simulink model "modeloNL1"  (R2025a)
settings: Solver=VariableStepAuto  StartTime=0.0  StopTime=100  FixedStep=0.01  RelTol=1e-3
undefined symbols (not defined in the file): C_alt, C_phi, C_theta, C_vel, INPUTS, Kp, Kp_sas, Kq, Kr, TrimInput, Xe
libraries: slpidlib x9
settings Model: Creator=anade  LastModifiedBy=Kaue

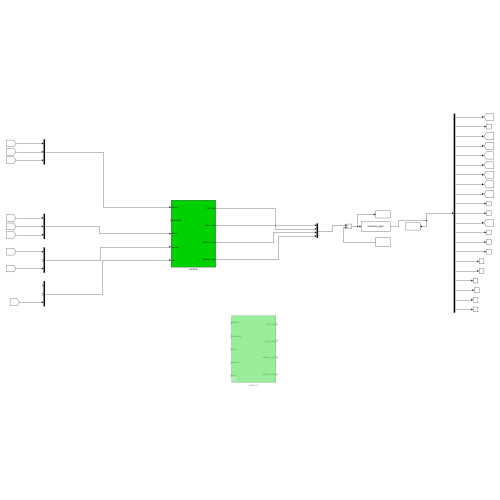
[thumbnail: Simulink's stored preview of the top-level diagram]
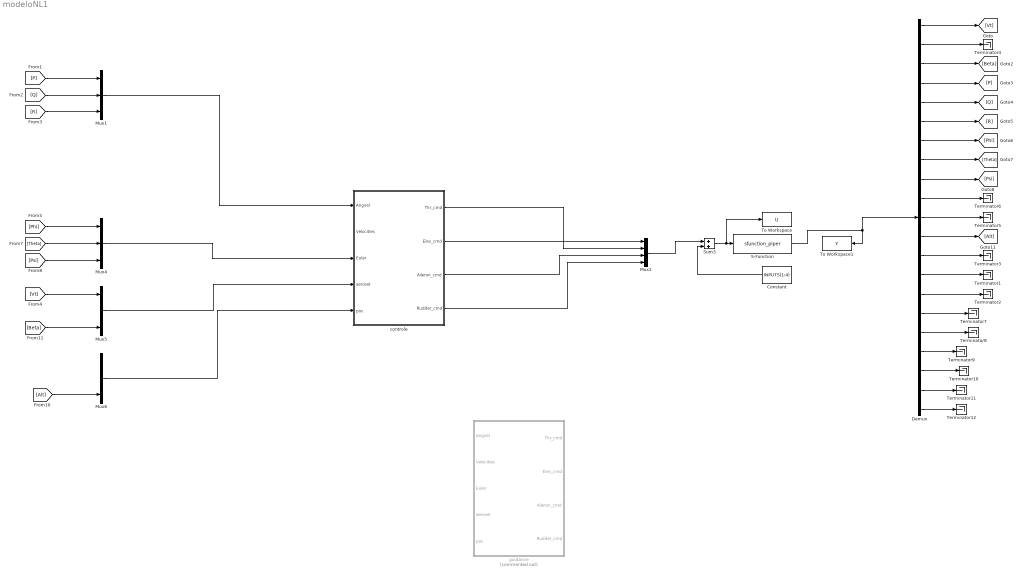
== system modeloNL1 ==
  Constant : Constant  Value=INPUTS(1:4)
  Demux : Demux  Outputs=21
  Mux{1,4..6} (4 alike) : Mux  Inputs=3
  Mux2 : Mux
  S-Function : S-Function  FunctionName=sfunction_piper  Parameters=par_gen,par_aero,par_prop, Xe  SFunctionDeploymentMode=off  EnableBusSupport=off
  Sum3 : Sum
  Terminator{1..12} (12 alike) : Terminator
  To Workspace : ToWorkspace  VariableName=U  SaveFormat=Structure With Time  SampleTime=-1
  To Workspace1 : ToWorkspace  VariableName=Y  SaveFormat=Structure With Time  SampleTime=-1
  controle : Subsystem
  guidance : Subsystem  Commented=on
  wires:
  S-Function/1 -> To Workspace1/1, Demux/1
  Sum3/1 -> To Workspace/1, S-Function/1
  controle/4(Rudder_cmd) -> Mux2/4
  controle/3(Aileron_cmd) -> Mux2/3
  Mux2/1 -> Sum3/1
  Constant/1 -> Sum3/2
  Demux/2 -> Terminator4/1
  Demux/3 -> [Beta]
  Demux/4 -> [P]
  Demux/5 -> [Q]
  Demux/6 -> [R]
  Demux/7 -> [Phi]
  Demux/8 -> [Theta]
  Demux/10 -> Terminator6/1
  Demux/11 -> Terminator5/1
  Demux/13 -> Terminator3/1
  Demux/14 -> Terminator1/1
  Demux/15 -> Terminator2/1
  Demux/1 -> [Vt]
  [Theta] -> Mux4/2
  Mux1/1 -> controle/1(Angvel)
  [Alt] -> Mux6/3
  [P] -> Mux1/1
  Mux4/1 -> controle/3(Euler)
  [R] -> Mux1/3
  [Phi] -> Mux4/1
  Mux6/1 -> controle/5(pos)
  [Q] -> Mux1/2
  Mux5/1 -> controle/4(aerovel)
  [Psi] -> Mux4/3
  [Beta] -> Mux5/3
  Demux/9 -> [Psi]
  [Vt] -> Mux5/1
  Demux/12 -> [Alt]
  controle/2(Elev_cmd) -> Mux2/1
  controle/1(Thr_cmd) -> Mux2/2
  Demux/17 -> Terminator8/1
  Demux/16 -> Terminator7/1
  Demux/19 -> Terminator10/1
  Demux/18 -> Terminator9/1
  Demux/21 -> Terminator12/1
  Demux/20 -> Terminator11/1

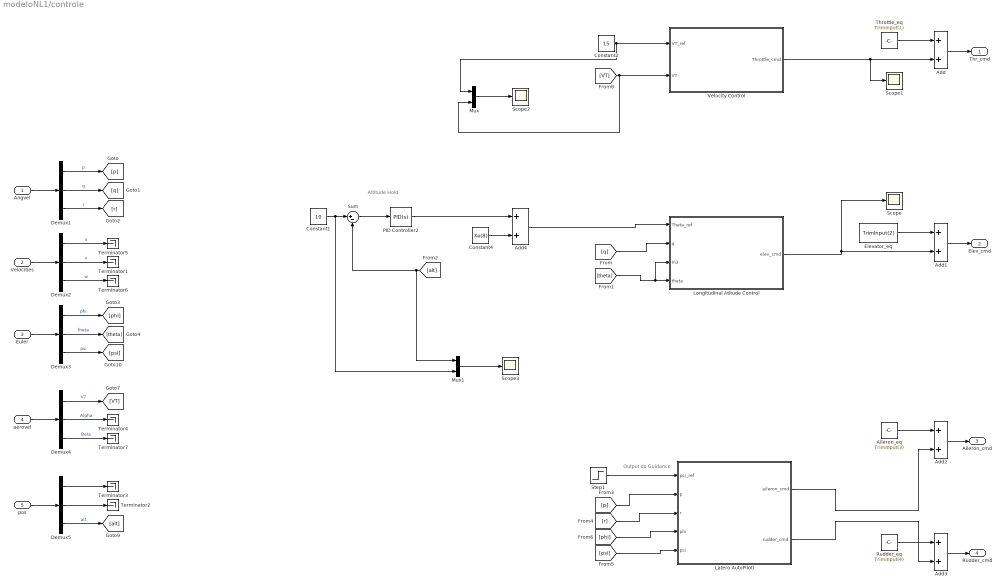
== system modeloNL1/controle ==
  note: Altitude Hold
  note: Output do Guidance
  Angvel : Inport
  Velocities : Inport  Port=2
  Euler : Inport  Port=3
  aerovel : Inport  Port=4
  pos : Inport  Port=5
  Add{,1..4} (5 alike) : Sum
  Aileron_eq : Constant  Value=TrimInput(3)
  Constant1 : Constant  Value=10
  Constant2 : Constant  Value=15
  Constant4 : Constant  Value=Xe(8)
  Demux{1..5} (5 alike) : Demux  Outputs=3
  Elevator_eq : Constant  Value=TrimInput(2)
  Latero AutoPilotl : Subsystem
  Longitudinal Atitude Control : Subsystem
  Mux : Mux  Inputs=2
  Mux1 : Mux  Inputs=2
  PID Controller2 : slpidlib/PID Controller  Controller=PID  Form=Parallel  TimeDomain=Continuous-time  UseExternalTs=off  SampleTime=-1  IntegratorMethod=Forward Euler  FilterMethod=Forward Euler  ControllerParametersSource=internal  P=C_alt.Kp  I=C_alt.Ki  UseKiTs=off  D=C_alt.Kd  UseExternalDerivativeSource=off  N=C_alt.N  UseFilter=on  TunerSelectOption=Transfer Function Based (PID Tuner App)  InitialConditionSource=internal  InitialConditionForIntegrator=0  InitialConditionForFilter=0  DifferentiatorICPrevScaledInput=0  ExternalReset=none  TrackingMode=off  Kt=1  LimitOutput=on  SatLimitsSource=internal  UpperSaturationLimit=0.26  LowerSaturationLimit=-0.17  LinearizeAsGain=on  AntiWindupMode=clamping  Kb=1  LimitIntegrator=off  UpperIntegratorSaturationLimit=inf  LowerIntegratorSaturationLimit=-inf  POutMin=[]  POutMax=[]  IOutMin=[]  IOutMax=[]  DOutMin=[]  DOutMax=[]  NOutMin=[]  NOutMax=[]  SumOutMin=[]  SumOutMax=[]  SaturationOutMin=[]  SaturationOutMax=[]  PParamMin=[]  PParamMax=[]  IParamMin=[]  IParamMax=[]  DParamMin=[]  DParamMax=[]  NParamMin=[]  NParamMax=[]  KbParamMin=[]  KbParamMax=[]  KtParamMin=[]  KtParamMax=[]  KbOutMin=[]  KbOutMax=[]  KtOutMin=[]  KtOutMax=[]  IntegratorOutMin=[]  IntegratorOutMax=[]  FilterOutMin=[]  FilterOutMax=[]  SumI1OutMin=[]  SumI1OutMax=[]  SumI2OutMin=[]  SumI2OutMax=[]  SumI3OutMin=[]  SumI3OutMax=[]  SumI4OutMin=[]  SumI4OutMax=[]  SumDOutMin=[]  SumDOutMax=[]  DifferentiatorOutMin=[]  DifferentiatorOutMax=[]  FilterDiffOutCoefMin=[]  FilterDiffOutCoefMax=[]  ReciprocalOutMin=[]  ReciprocalOutMax=[]  SumDenOutMin=[]  SumDenOutMax=[]  SumNumOutMin=[]  SumNumOutMax=[]  DivideOutMin=[]  DivideOutMax=[]  UdiffTsProdOutMin=[]  UdiffTsProdOutMax=[]  NTsProdOutMin=[]  NTsProdOutMax=[]  UintegralTsProdOutMin=[]  UintegralTsProdOutMax=[]  UngainTsProdOutMin=[]  UngainTsProdOutMax=[]  ClampingZeroOutDataTypeStr=Inherit: Inherit via back propagation  ClampingZeroOutMin=[]  ClampingZeroOutMax=[]  FilterDenConstantOutDataTypeStr=Inherit: Inherit via back propagation  FilterDenConstantOutMin=[]  FilterDenConstantOutMax=[]  PCopyOutDataTypeStr=Inherit: Inherit via back propagation  PCopyOutMin=[]  PCopyOutMax=[]  NCopyOutDataTypeStr=Inherit: Inherit via back propagation  NCopyOutMin=[]  NCopyOutMax=[]  IntegratorContinuousStateAttributes=''  IntegratorStateMustResolveToSignalObject=off  IntegratorRTWStateStorageClass=Auto  FilterContinuousStateAttributes=''  FilterStateMustResolveToSignalObject=off  FilterRTWStateStorageClass=Auto  ParallelPVariant=InternalParameters  IdealPVariant=Disabled  IVariant=InternalParameters  DVariant=InternalParameters  IntegratorVariant=Continuous  SatVariant=Enabled  AWVariant=ContClampingParallel  PCopyVariant=Disabled  TRVariant=Disabled  FdbkBlocksVariant=Forward  IdealPFdbkVariant=Disabled  SatFdbkVariant=Disabled  DerivativeFilterVariant=ContFilter  NVariant=InternalParameters  NCopyVariant=Disabled  FilterICVariant=InternalICsFilter  IntegratorICVariant=InternalICs  ExternalResetVariant=Disabled  TRSumVariant=Passthrough  SumFdbkVariant=Disabled  SumVariant=Sum_PID  TsampFilterVariant=InternalTs  TsampNgainVariant=Passthrough  TsampIntegralVariant=Disabled_SignalSpec  ExternalSaturationOutDataTypeStr=Inherit: Same as second input  DerivativeSourceVariant=ErrorSignal  PreIntVariant=InternalPreInt
  Rudder_eq : Constant  Value=TrimInput(4)
  Scope{,1..3} (4 alike) : Scope
      Scope settings: ActiveDisplayYMinimum=-1E-5  ActiveDisplayYMaximum=0.0001
      Scope1 settings: ActiveDisplayYMinimum=-746.9186  ActiveDisplayYMaximum=116.1605  DataLoggingVariableName=ScopeData2
      Scope2 settings: ActiveDisplayYMinimum=-99.881928520684582  ActiveDisplayYMaximum=101.11428639075469  DataLoggingVariableName=ScopeData4
      Scope3 settings: ActiveDisplayYMinimum=-113.29137312954269  ActiveDisplayYMaximum=148.47510576001991  DataLoggingVariableName=ScopeData6
  Step1 : Step  Time=5  After=deg2rad(45)  SampleTime=0
  Sum : Sum  Inputs=|+-
  Terminator{1..7} (7 alike) : Terminator
  Throttle_eq : Constant  Value=TrimInput(1)
  Velocity Control : Subsystem
  Thr_cmd : Outport
  Elev_cmd : Outport  Port=2
  Aileron_cmd : Outport  Port=3
  Rudder_cmd : Outport  Port=4
  wires:
  Angvel/1 -> Demux1/1
  Velocities/1 -> Demux2/1
  Demux1/1 -> [p]  "p"
  Demux1/2 -> [q]  "q"
  Demux1/3 -> [r]  "r"
  Euler/1 -> Demux3/1
  Demux3/3 -> [psi]  "psi"
  Demux3/1 -> [phi]  "phi"
  Demux3/2 -> [theta]  "theta"
  Demux2/3 -> Terminator6/1  "w"
  Demux2/1 -> Terminator5/1  "u"
  Demux2/2 -> Terminator1/1  "v"
  [theta] -> Longitudinal Atitude Control/3(In3), Longitudinal Atitude Control/4(theta)
  aerovel/1 -> Demux4/1
  Demux4/1 -> [VT]  "VT"
  Demux4/2 -> Terminator4/1  "Alpha"
  Demux4/3 -> Terminator7/1  "Beta"
  [q] -> Longitudinal Atitude Control/2(q)
  [VT] -> Mux/2, Velocity Control/2(VT)
  pos/1 -> Demux5/1
  Demux5/3 -> [alt]  "alt"
  Demux5/2 -> Terminator2/1
  Demux5/1 -> Terminator3/1
  [alt] -> Sum/2, Mux1/1
  [p] -> Latero AutoPilotl/2(p)
  [r] -> Latero AutoPilotl/3(r)
  [psi] -> Latero AutoPilotl/5(psi)
  [phi] -> Latero AutoPilotl/4(phi)
  Constant4/1 -> Add4/2
  Add4/1 -> Longitudinal Atitude Control/1(Theta_ref)
  Step1/1 -> Latero AutoPilotl/1(psi_ref)
  Constant1/1 -> Mux1/2, Sum/1
  Mux/1 -> Scope2/1
  Add1/1 -> Elev_cmd/1
  Longitudinal Atitude Control/1(elev_cmd) -> Scope/1, Add1/2
  Add/1 -> Thr_cmd/1
  Velocity Control/1(Throttle_cmd) -> Scope1/1, Add/2
  Latero AutoPilotl/1(aileron_cmd) -> Add2/2
  Elevator_eq/1 -> Add1/1
  Rudder_eq/1 -> Add3/1
  Aileron_eq/1 -> Add2/1
  Latero AutoPilotl/2(rudder_cmd) -> Add3/2
  Add2/1 -> Aileron_cmd/1
  Add3/1 -> Rudder_cmd/1
  Throttle_eq/1 -> Add/1
  Mux1/1 -> Scope3/1
  Sum/1 -> PID Controller2/1
  PID Controller2/1 -> Add4/1
  Constant2/1 -> Mux/1, Velocity Control/1(VT_ref)

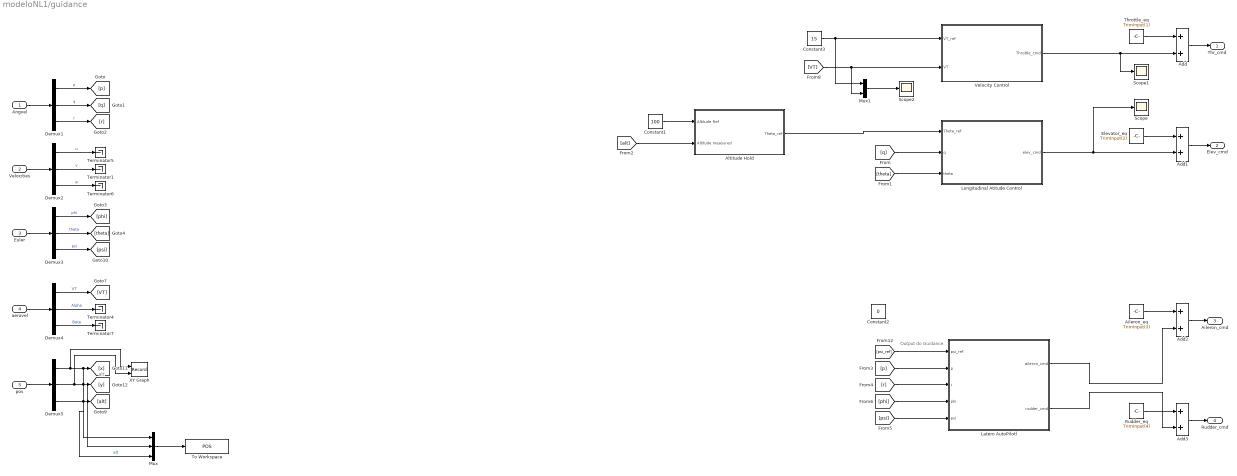
== system modeloNL1/guidance ==
  note: alt
  note: Output do Guidance
  Angvel : Inport
  Velocities : Inport  Port=2
  Euler : Inport  Port=3
  aerovel : Inport  Port=4
  pos : Inport  Port=5
  Add{,1..3} (4 alike) : Sum
  Aileron_eq : Constant  Value=TrimInput(3)
  Altitude Hold : Subsystem
  Constant1 : Constant  Value=100
  Constant2 : Constant  Value=0
  Constant3 : Constant  Value=15
  Demux{1..5} (5 alike) : Demux  Outputs=3
  Elevator_eq : Constant  Value=TrimInput(2)
  Latero AutoPilotl : Subsystem
  Longitudinal Atitude Control : Subsystem
  Mux : Mux  Inputs=3
  Mux1 : Mux  Inputs=2
  Rudder_eq : Constant  Value=TrimInput(4)
  Scope : Scope
      settings: ActiveDisplayYMinimum=-0.12211  ActiveDisplayYMaximum=0.19601
  Scope1 : Scope
      settings: ActiveDisplayYMinimum=-0.14231  ActiveDisplayYMaximum=0.53618  DataLoggingVariableName=ScopeData2
  Scope2 : Scope
      settings: ActiveDisplayYMinimum=-393.97180191646771  ActiveDisplayYMaximum=165.99613363913147
  Terminator{1,4..7} (5 alike) : Terminator
  Throttle_eq : Constant  Value=TrimInput(1)
  To Workspace : ToWorkspace  VariableName=POS  SaveFormat=Timeseries  SampleTime=-1
  Velocity Control : Subsystem
  XY Graph : Record  NumPorts=2.0  FileSettingsInternal="{\"entries\":[{\"content\":{\"excelSettings\":{\"content\":{},\"type\":\"Streamout.ExcelSettings\"},\"parquetSettings\":{\"content\":{},\"type\":\"Streamout.ParquetSettings\"}},\"type\":\"Streamout.FileSettingStorage\",\"uuid\":\"\"}],\"packageUris\":[\"http:\\/\\/schema.mathworks.com\\/mf0\\/streamout_blocks\\/R2020a\"],\"version\":\"1.0\"}"  FrameSettings=[0, 0]  Layout=[1 1]  SignalsInternal="{\"entries\":[{\"content\":{\"signals\":[{\"content\":{\"blockPath\":[],\"dimensions\":[1],\"domain\":\"\",\"lineColor\":\"#a2142f\",\"plots\":[ 1 ],\"port\":1,\"signalID\":1,\"signalName\":\"Demux5:1\"},\"type\":\"RecordBlkView.Signal\",\"uuid\":\"\"},{\"content\":{\"blockPath\":[],\"dimensions\":[1],\"domain\":\"\",\"lineColor\":\"#139fff\",\"plots\":[ 1 ],\"port\":2,\"signalID\":2,\"signalName\":\"Demux5:2\"},\"type\":\"RecordBlkView.Signal\",\"uuid\":\"\"}]},\"type\":\"RecordBlkView.InputSignals\",\"uuid\":\"\"}],\"packageUris\":[\"http:\\/\\/schema.mathworks.com\\/mf0\\/streamout_blocks\\/R2020a\"],\"version\":\"1.0\"}"  VisualizationBindings="{\"xyplotplugin\":{\"info\":[{\"series\":[{\"bindingParametersList\":[{\"parameter\":\"X-Axis\",\"signalID\":1,\"signalName\":\"Demux5:1\"},{\"parameter\":\"Y-Axis\",\"signalID\":2,\"signalName\":\"Demux5:2\"}],\"seriesID\":0}],\"subplotID\":1}]}}"  CompatibilityTag=XY
  Thr_cmd : Outport
  Elev_cmd : Outport  Port=2
  Aileron_cmd : Outport  Port=3
  Rudder_cmd : Outport  Port=4
  wires:
  Angvel/1 -> Demux1/1
  Velocities/1 -> Demux2/1
  Demux1/1 -> [p]  "p"
  Demux1/2 -> [q]  "q"
  Demux1/3 -> [r]  "r"
  Euler/1 -> Demux3/1
  Demux3/3 -> [psi]  "psi"
  Demux3/1 -> [phi]  "phi"
  Demux3/2 -> [theta]  "theta"
  Demux2/3 -> Terminator6/1  "w"
  Demux2/1 -> Terminator5/1  "u"
  Demux2/2 -> Terminator1/1  "v"
  [theta] -> Longitudinal Atitude Control/3(theta)
  aerovel/1 -> Demux4/1
  Demux4/1 -> [VT]  "VT"
  Demux4/2 -> Terminator4/1  "Alpha"
  Demux4/3 -> Terminator7/1  "Beta"
  Add/1 -> Thr_cmd/1
  Add2/1 -> Aileron_cmd/1
  Add3/1 -> Rudder_cmd/1
  Throttle_eq/1 -> Add/1
  Aileron_eq/1 -> Add2/1
  Rudder_eq/1 -> Add3/1
  [q] -> Longitudinal Atitude Control/2(q)
  Elevator_eq/1 -> Add1/1
  Add1/1 -> Elev_cmd/1
  Longitudinal Atitude Control/1(elev_cmd) -> Scope/1, Add1/2
  [VT] -> Velocity Control/2(VT), Mux1/2
  pos/1 -> Demux5/1
  Demux5/3 -> Mux/3, [alt]  "alt"
  Demux5/2 -> XY Graph/2, Mux/2, [y]
  Latero AutoPilotl/1(aileron_cmd) -> Add2/2
  Latero AutoPilotl/2(rudder_cmd) -> Add3/2
  [p] -> Latero AutoPilotl/2(p)
  [r] -> Latero AutoPilotl/3(r)
  [psi] -> Latero AutoPilotl/5(psi)
  [phi] -> Latero AutoPilotl/4(phi)
  Constant3/1 -> Mux1/1, Velocity Control/1(VT_ref)
  Velocity Control/1(Throttle_cmd) -> Scope1/1, Add/2
  Altitude Hold/1(Theta_ref) -> Longitudinal Atitude Control/1(Theta_ref)
  [alt] -> Altitude Hold/2(Altitude measured)
  Constant1/1 -> Altitude Hold/1(Altitude Ref)
  [psi_ref] -> Latero AutoPilotl/1(psi_ref)
  Demux5/1 -> XY Graph/1, Mux/1, [x]
  Mux/1 -> To Workspace/1
  Mux1/1 -> Scope2/1

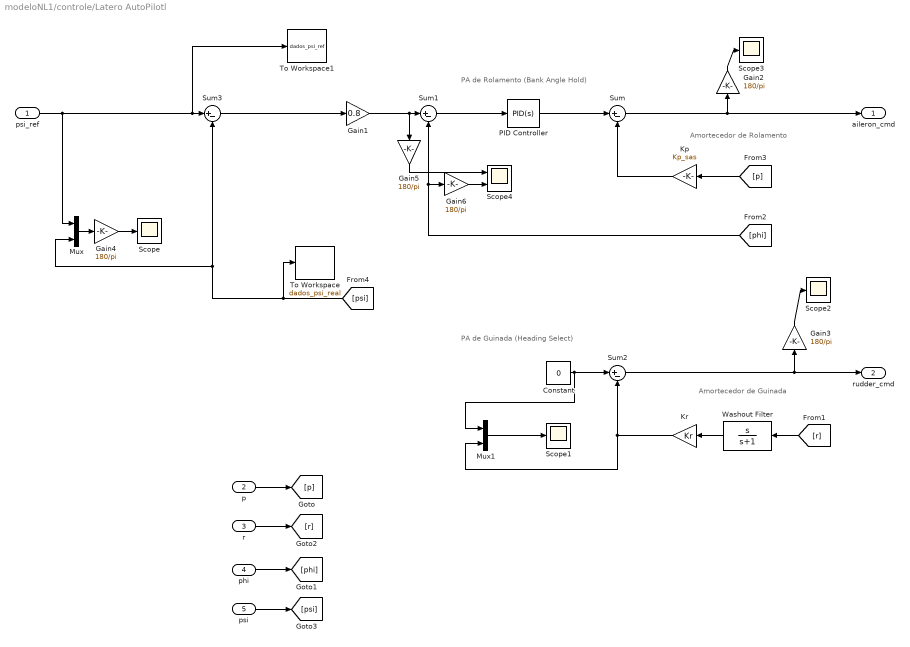
== system modeloNL1/controle/Latero AutoPilotl ==
  note: PA de Rolamento (Bank Angle Hold)
  note: Amortecedor de Rolamento
  note: Amortecedor de Guinada
  note: PA de Guinada (Heading Select)
  psi_ref : Inport
  p : Inport  Port=2
  r : Inport  Port=3
  phi : Inport  Port=4
  psi : Inport  Port=5
  Constant : Constant  Value=0
  Gain1 : Gain  Gain=0.8
  Gain{2..6} (5 alike) : Gain  Gain=180/pi
  Kp : Gain  Gain=Kp_sas
  Kr : Gain  Gain=Kr
  Mux : Mux  Inputs=2
  Mux1 : Mux  Inputs=2
  PID Controller : slpidlib/PID Controller  Controller=PID  Form=Parallel  TimeDomain=Continuous-time  UseExternalTs=off  SampleTime=-1  IntegratorMethod=Forward Euler  FilterMethod=Forward Euler  ControllerParametersSource=internal  P=C_phi.Kp  I=C_phi.Ki  UseKiTs=off  D=C_phi.Kd  UseExternalDerivativeSource=off  N=C_phi.N  UseFilter=on  TunerSelectOption=Transfer Function Based (PID Tuner App)  InitialConditionSource=internal  InitialConditionForIntegrator=0  InitialConditionForFilter=0  DifferentiatorICPrevScaledInput=0  ExternalReset=none  TrackingMode=off  Kt=1  LimitOutput=off  SatLimitsSource=internal  UpperSaturationLimit=inf  LowerSaturationLimit=-inf  LinearizeAsGain=on  AntiWindupMode=none  Kb=1  LimitIntegrator=off  UpperIntegratorSaturationLimit=inf  LowerIntegratorSaturationLimit=-inf  POutMin=[]  POutMax=[]  IOutMin=[]  IOutMax=[]  DOutMin=[]  DOutMax=[]  NOutMin=[]  NOutMax=[]  SumOutMin=[]  SumOutMax=[]  SaturationOutMin=[]  SaturationOutMax=[]  PParamMin=[]  PParamMax=[]  IParamMin=[]  IParamMax=[]  DParamMin=[]  DParamMax=[]  NParamMin=[]  NParamMax=[]  KbParamMin=[]  KbParamMax=[]  KtParamMin=[]  KtParamMax=[]  KbOutMin=[]  KbOutMax=[]  KtOutMin=[]  KtOutMax=[]  IntegratorOutMin=[]  IntegratorOutMax=[]  FilterOutMin=[]  FilterOutMax=[]  SumI1OutMin=[]  SumI1OutMax=[]  SumI2OutMin=[]  SumI2OutMax=[]  SumI3OutMin=[]  SumI3OutMax=[]  SumI4OutMin=[]  SumI4OutMax=[]  SumDOutMin=[]  SumDOutMax=[]  DifferentiatorOutMin=[]  DifferentiatorOutMax=[]  FilterDiffOutCoefMin=[]  FilterDiffOutCoefMax=[]  ReciprocalOutMin=[]  ReciprocalOutMax=[]  SumDenOutMin=[]  SumDenOutMax=[]  SumNumOutMin=[]  SumNumOutMax=[]  DivideOutMin=[]  DivideOutMax=[]  UdiffTsProdOutMin=[]  UdiffTsProdOutMax=[]  NTsProdOutMin=[]  NTsProdOutMax=[]  UintegralTsProdOutMin=[]  UintegralTsProdOutMax=[]  UngainTsProdOutMin=[]  UngainTsProdOutMax=[]  ClampingZeroOutDataTypeStr=Inherit: Inherit via back propagation  ClampingZeroOutMin=[]  ClampingZeroOutMax=[]  FilterDenConstantOutDataTypeStr=Inherit: Inherit via back propagation  FilterDenConstantOutMin=[]  FilterDenConstantOutMax=[]  PCopyOutDataTypeStr=Inherit: Inherit via back propagation  PCopyOutMin=[]  PCopyOutMax=[]  NCopyOutDataTypeStr=Inherit: Inherit via back propagation  NCopyOutMin=[]  NCopyOutMax=[]  IntegratorContinuousStateAttributes=''  IntegratorStateMustResolveToSignalObject=off  IntegratorRTWStateStorageClass=Auto  FilterContinuousStateAttributes=''  FilterStateMustResolveToSignalObject=off  FilterRTWStateStorageClass=Auto  ParallelPVariant=InternalParameters  IdealPVariant=Disabled  IVariant=InternalParameters  DVariant=InternalParameters  IntegratorVariant=Continuous  SatVariant=Disabled  AWVariant=Passthrough  PCopyVariant=Disabled  TRVariant=Disabled  FdbkBlocksVariant=Forward  IdealPFdbkVariant=Disabled  SatFdbkVariant=Disabled  DerivativeFilterVariant=ContFilter  NVariant=InternalParameters  NCopyVariant=Disabled  FilterICVariant=InternalICsFilter  IntegratorICVariant=InternalICs  ExternalResetVariant=Disabled  TRSumVariant=Passthrough  SumFdbkVariant=Disabled  SumVariant=Sum_PID  TsampFilterVariant=InternalTs  TsampNgainVariant=Passthrough  TsampIntegralVariant=Disabled_SignalSpec  ExternalSaturationOutDataTypeStr=Inherit: Same as second input  DerivativeSourceVariant=ErrorSignal  PreIntVariant=InternalPreInt
  Scope{,1..3} (4 alike) : Scope
      Scope settings: ActiveDisplayYMinimum=-9.73683  ActiveDisplayYMaximum=51.08187  DataLoggingVariableName=ScopeData5
      Scope1 settings: ActiveDisplayYMinimum=-0.64466  ActiveDisplayYMaximum=0.29284
      Scope2 settings: ActiveDisplayYMinimum=-4.64142  ActiveDisplayYMaximum=2.08449
      Scope3 settings: ActiveDisplayYMinimum=-384.74036  ActiveDisplayYMaximum=1108.75141  DataLoggingVariableName=ScopeData2
  Scope4 : Scope  NumInputPorts=2
      settings: ActiveDisplayYMinimum=-4.8655  ActiveDisplayYMaximum=43.78946  DataLoggingVariableName=ScopeData3
  Sum{,1..3} (4 alike) : Sum  Inputs=|+-
  To Workspace : ToWorkspace  VariableName=dados_psi_real  SaveFormat=Timeseries  SampleTime=-1
      settings: Save2DSignal=2-D array (concatenate along first dimension)
  To Workspace1 : ToWorkspace  VariableName=dados_psi_ref  SaveFormat=Timeseries  SampleTime=-1
      settings: Save2DSignal=2-D array (concatenate along first dimension)
  Washout Filter : TransferFcn  Numerator=[1 0]  Denominator=[1 1]
  aileron_cmd : Outport
  rudder_cmd : Outport  Port=2
  wires:
  Sum1/1 -> PID Controller/1
  Sum/1 -> Gain2/1, aileron_cmd/1
  [p] -> Kp/1
  [phi] -> Sum1/2, Gain6/1
  Kp/1 -> Sum/2
  PID Controller/1 -> Sum/1
  p/1 -> [p]
  [r] -> Washout Filter/1
  Kr/1 -> Mux1/2, Sum2/2
  r/1 -> [r]
  Washout Filter/1 -> Kr/1
  phi/1 -> [phi]
  psi/1 -> [psi]
  Sum3/1 -> Gain1/1
  [psi] -> To Workspace/1, Sum3/2, Mux/2
  psi_ref/1 -> Mux/1, To Workspace1/1, Sum3/1
  Sum2/1 -> Gain3/1, rudder_cmd/1
  Constant/1 -> Mux1/1, Sum2/1
  Gain1/1 -> Gain5/1, Sum1/1
  Mux/1 -> Gain4/1
  Mux1/1 -> Scope1/1
  Gain2/1 -> Scope3/1
  Gain3/1 -> Scope2/1
  Gain4/1 -> Scope/1
  Gain5/1 -> Scope4/1
  Gain6/1 -> Scope4/2

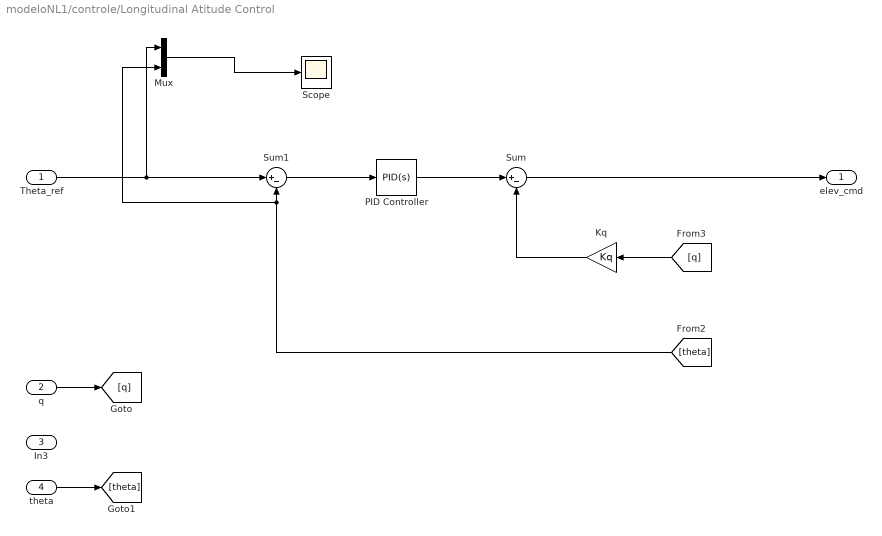
== system modeloNL1/controle/Longitudinal Atitude Control ==
  Theta_ref : Inport
  q : Inport  Port=2
  In3 : Inport  Port=3
  theta : Inport  Port=4
  Kq : Gain  Gain=Kq
  Mux : Mux  Inputs=2
  PID Controller : slpidlib/PID Controller  Controller=PID  Form=Parallel  TimeDomain=Continuous-time  UseExternalTs=off  SampleTime=-1  IntegratorMethod=Forward Euler  FilterMethod=Forward Euler  ControllerParametersSource=internal  P=C_theta.Kp  I=C_theta.Ki  UseKiTs=off  D=C_theta.Kd  UseExternalDerivativeSource=off  N=C_theta.N  UseFilter=on  TunerSelectOption=Transfer Function Based (PID Tuner App)  InitialConditionSource=internal  InitialConditionForIntegrator=0  InitialConditionForFilter=0  DifferentiatorICPrevScaledInput=0  ExternalReset=none  TrackingMode=off  Kt=1  LimitOutput=off  SatLimitsSource=internal  UpperSaturationLimit=inf  LowerSaturationLimit=-inf  LinearizeAsGain=on  AntiWindupMode=none  Kb=1  LimitIntegrator=off  UpperIntegratorSaturationLimit=inf  LowerIntegratorSaturationLimit=-inf  POutMin=[]  POutMax=[]  IOutMin=[]  IOutMax=[]  DOutMin=[]  DOutMax=[]  NOutMin=[]  NOutMax=[]  SumOutMin=[]  SumOutMax=[]  SaturationOutMin=[]  SaturationOutMax=[]  PParamMin=[]  PParamMax=[]  IParamMin=[]  IParamMax=[]  DParamMin=[]  DParamMax=[]  NParamMin=[]  NParamMax=[]  KbParamMin=[]  KbParamMax=[]  KtParamMin=[]  KtParamMax=[]  KbOutMin=[]  KbOutMax=[]  KtOutMin=[]  KtOutMax=[]  IntegratorOutMin=[]  IntegratorOutMax=[]  FilterOutMin=[]  FilterOutMax=[]  SumI1OutMin=[]  SumI1OutMax=[]  SumI2OutMin=[]  SumI2OutMax=[]  SumI3OutMin=[]  SumI3OutMax=[]  SumI4OutMin=[]  SumI4OutMax=[]  SumDOutMin=[]  SumDOutMax=[]  DifferentiatorOutMin=[]  DifferentiatorOutMax=[]  FilterDiffOutCoefMin=[]  FilterDiffOutCoefMax=[]  ReciprocalOutMin=[]  ReciprocalOutMax=[]  SumDenOutMin=[]  SumDenOutMax=[]  SumNumOutMin=[]  SumNumOutMax=[]  DivideOutMin=[]  DivideOutMax=[]  UdiffTsProdOutMin=[]  UdiffTsProdOutMax=[]  NTsProdOutMin=[]  NTsProdOutMax=[]  UintegralTsProdOutMin=[]  UintegralTsProdOutMax=[]  UngainTsProdOutMin=[]  UngainTsProdOutMax=[]  ClampingZeroOutDataTypeStr=Inherit: Inherit via back propagation  ClampingZeroOutMin=[]  ClampingZeroOutMax=[]  FilterDenConstantOutDataTypeStr=Inherit: Inherit via back propagation  FilterDenConstantOutMin=[]  FilterDenConstantOutMax=[]  PCopyOutDataTypeStr=Inherit: Inherit via back propagation  PCopyOutMin=[]  PCopyOutMax=[]  NCopyOutDataTypeStr=Inherit: Inherit via back propagation  NCopyOutMin=[]  NCopyOutMax=[]  IntegratorContinuousStateAttributes=''  IntegratorStateMustResolveToSignalObject=off  IntegratorRTWStateStorageClass=Auto  FilterContinuousStateAttributes=''  FilterStateMustResolveToSignalObject=off  FilterRTWStateStorageClass=Auto  ParallelPVariant=InternalParameters  IdealPVariant=Disabled  IVariant=InternalParameters  DVariant=InternalParameters  IntegratorVariant=Continuous  SatVariant=Disabled  AWVariant=Passthrough  PCopyVariant=Disabled  TRVariant=Disabled  FdbkBlocksVariant=Forward  IdealPFdbkVariant=Disabled  SatFdbkVariant=Disabled  DerivativeFilterVariant=ContFilter  NVariant=InternalParameters  NCopyVariant=Disabled  FilterICVariant=InternalICsFilter  IntegratorICVariant=InternalICs  ExternalResetVariant=Disabled  TRSumVariant=Passthrough  SumFdbkVariant=Disabled  SumVariant=Sum_PID  TsampFilterVariant=InternalTs  TsampNgainVariant=Passthrough  TsampIntegralVariant=Disabled_SignalSpec  ExternalSaturationOutDataTypeStr=Inherit: Same as second input  DerivativeSourceVariant=ErrorSignal  PreIntVariant=InternalPreInt
  Scope : Scope
      settings: ActiveDisplayYMinimum=-0.22285  ActiveDisplayYMaximum=0.02179  DataLoggingVariableName=ScopeData3
  Sum : Sum  Inputs=|+-
  Sum1 : Sum  Inputs=|+-
  elev_cmd : Outport
  wires:
  Sum1/1 -> PID Controller/1
  Sum/1 -> elev_cmd/1
  [q] -> Kq/1
  [theta] -> Mux/2, Sum1/2
  Kq/1 -> Sum/2
  PID Controller/1 -> Sum/1
  theta/1 -> [theta]
  q/1 -> [q]
  Theta_ref/1 -> Mux/1, Sum1/1
  Mux/1 -> Scope/1

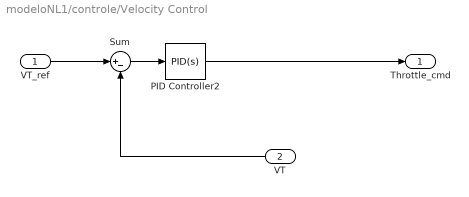
== system modeloNL1/controle/Velocity Control ==
  VT_ref : Inport
  VT : Inport  Port=2
  PID Controller2 : slpidlib/PID Controller  Controller=PID  Form=Parallel  TimeDomain=Continuous-time  UseExternalTs=off  SampleTime=-1  IntegratorMethod=Forward Euler  FilterMethod=Forward Euler  ControllerParametersSource=internal  P=-C_vel.Kp  I=-C_vel.Ki  UseKiTs=off  D=-C_vel.Kd  UseExternalDerivativeSource=off  N=C_vel.N  UseFilter=on  TunerSelectOption=Transfer Function Based (PID Tuner App)  InitialConditionSource=internal  InitialConditionForIntegrator=0  InitialConditionForFilter=0  DifferentiatorICPrevScaledInput=0  ExternalReset=none  TrackingMode=off  Kt=1  LimitOutput=off  SatLimitsSource=internal  UpperSaturationLimit=inf  LowerSaturationLimit=-inf  LinearizeAsGain=on  AntiWindupMode=none  Kb=1  LimitIntegrator=off  UpperIntegratorSaturationLimit=inf  LowerIntegratorSaturationLimit=-inf  POutMin=[]  POutMax=[]  IOutMin=[]  IOutMax=[]  DOutMin=[]  DOutMax=[]  NOutMin=[]  NOutMax=[]  SumOutMin=[]  SumOutMax=[]  SaturationOutMin=[]  SaturationOutMax=[]  PParamMin=[]  PParamMax=[]  IParamMin=[]  IParamMax=[]  DParamMin=[]  DParamMax=[]  NParamMin=[]  NParamMax=[]  KbParamMin=[]  KbParamMax=[]  KtParamMin=[]  KtParamMax=[]  KbOutMin=[]  KbOutMax=[]  KtOutMin=[]  KtOutMax=[]  IntegratorOutMin=[]  IntegratorOutMax=[]  FilterOutMin=[]  FilterOutMax=[]  SumI1OutMin=[]  SumI1OutMax=[]  SumI2OutMin=[]  SumI2OutMax=[]  SumI3OutMin=[]  SumI3OutMax=[]  SumI4OutMin=[]  SumI4OutMax=[]  SumDOutMin=[]  SumDOutMax=[]  DifferentiatorOutMin=[]  DifferentiatorOutMax=[]  FilterDiffOutCoefMin=[]  FilterDiffOutCoefMax=[]  ReciprocalOutMin=[]  ReciprocalOutMax=[]  SumDenOutMin=[]  SumDenOutMax=[]  SumNumOutMin=[]  SumNumOutMax=[]  DivideOutMin=[]  DivideOutMax=[]  UdiffTsProdOutMin=[]  UdiffTsProdOutMax=[]  NTsProdOutMin=[]  NTsProdOutMax=[]  UintegralTsProdOutMin=[]  UintegralTsProdOutMax=[]  UngainTsProdOutMin=[]  UngainTsProdOutMax=[]  ClampingZeroOutDataTypeStr=Inherit: Inherit via back propagation  ClampingZeroOutMin=[]  ClampingZeroOutMax=[]  FilterDenConstantOutDataTypeStr=Inherit: Inherit via back propagation  FilterDenConstantOutMin=[]  FilterDenConstantOutMax=[]  PCopyOutDataTypeStr=Inherit: Inherit via back propagation  PCopyOutMin=[]  PCopyOutMax=[]  NCopyOutDataTypeStr=Inherit: Inherit via back propagation  NCopyOutMin=[]  NCopyOutMax=[]  IntegratorContinuousStateAttributes=''  IntegratorStateMustResolveToSignalObject=off  IntegratorRTWStateStorageClass=Auto  FilterContinuousStateAttributes=''  FilterStateMustResolveToSignalObject=off  FilterRTWStateStorageClass=Auto  ParallelPVariant=InternalParameters  IdealPVariant=Disabled  IVariant=InternalParameters  DVariant=InternalParameters  IntegratorVariant=Continuous  SatVariant=Disabled  AWVariant=Passthrough  PCopyVariant=Disabled  TRVariant=Disabled  FdbkBlocksVariant=Forward  IdealPFdbkVariant=Disabled  SatFdbkVariant=Disabled  DerivativeFilterVariant=ContFilter  NVariant=InternalParameters  NCopyVariant=Disabled  FilterICVariant=InternalICsFilter  IntegratorICVariant=InternalICs  ExternalResetVariant=Disabled  TRSumVariant=Passthrough  SumFdbkVariant=Disabled  SumVariant=Sum_PID  TsampFilterVariant=InternalTs  TsampNgainVariant=Passthrough  TsampIntegralVariant=Disabled_SignalSpec  ExternalSaturationOutDataTypeStr=Inherit: Same as second input  DerivativeSourceVariant=ErrorSignal  PreIntVariant=InternalPreInt
  Sum : Sum  Inputs=|+-
  Throttle_cmd : Outport
  wires:
  VT/1 -> Sum/2
  PID Controller2/1 -> Throttle_cmd/1
  VT_ref/1 -> Sum/1
  Sum/1 -> PID Controller2/1

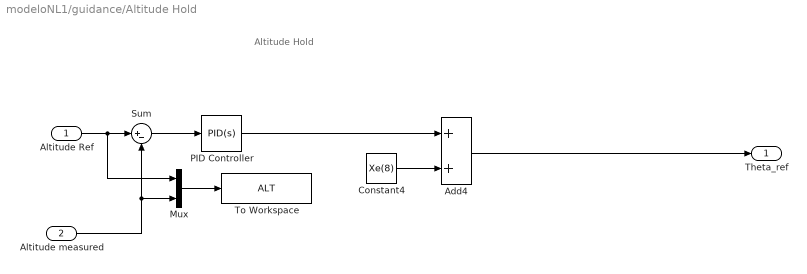
== system modeloNL1/guidance/Altitude Hold ==
  note: Altitude Hold
  Altitude Ref : Inport
  Altitude measured : Inport  Port=2
  Add4 : Sum
  Constant4 : Constant  Value=Xe(8)
  Mux : Mux  Inputs=2
  PID Controller : slpidlib/PID Controller  Controller=PID  Form=Parallel  TimeDomain=Continuous-time  UseExternalTs=off  SampleTime=-1  IntegratorMethod=Forward Euler  FilterMethod=Forward Euler  ControllerParametersSource=internal  P=C_alt.Kp  I=C_alt.Ki  UseKiTs=off  D=C_alt.Kd  UseExternalDerivativeSource=off  N=C_alt.N  UseFilter=on  TunerSelectOption=Transfer Function Based (PID Tuner App)  InitialConditionSource=internal  InitialConditionForIntegrator=0  InitialConditionForFilter=0  DifferentiatorICPrevScaledInput=0  ExternalReset=none  TrackingMode=off  Kt=1  LimitOutput=on  SatLimitsSource=internal  UpperSaturationLimit=0.26  LowerSaturationLimit=-0.17  LinearizeAsGain=on  AntiWindupMode=back-calculation  Kb=1  LimitIntegrator=off  UpperIntegratorSaturationLimit=inf  LowerIntegratorSaturationLimit=-inf  POutMin=[]  POutMax=[]  IOutMin=[]  IOutMax=[]  DOutMin=[]  DOutMax=[]  NOutMin=[]  NOutMax=[]  SumOutMin=[]  SumOutMax=[]  SaturationOutMin=[]  SaturationOutMax=[]  PParamMin=[]  PParamMax=[]  IParamMin=[]  IParamMax=[]  DParamMin=[]  DParamMax=[]  NParamMin=[]  NParamMax=[]  KbParamMin=[]  KbParamMax=[]  KtParamMin=[]  KtParamMax=[]  KbOutMin=[]  KbOutMax=[]  KtOutMin=[]  KtOutMax=[]  IntegratorOutMin=[]  IntegratorOutMax=[]  FilterOutMin=[]  FilterOutMax=[]  SumI1OutMin=[]  SumI1OutMax=[]  SumI2OutMin=[]  SumI2OutMax=[]  SumI3OutMin=[]  SumI3OutMax=[]  SumI4OutMin=[]  SumI4OutMax=[]  SumDOutMin=[]  SumDOutMax=[]  DifferentiatorOutMin=[]  DifferentiatorOutMax=[]  FilterDiffOutCoefMin=[]  FilterDiffOutCoefMax=[]  ReciprocalOutMin=[]  ReciprocalOutMax=[]  SumDenOutMin=[]  SumDenOutMax=[]  SumNumOutMin=[]  SumNumOutMax=[]  DivideOutMin=[]  DivideOutMax=[]  UdiffTsProdOutMin=[]  UdiffTsProdOutMax=[]  NTsProdOutMin=[]  NTsProdOutMax=[]  UintegralTsProdOutMin=[]  UintegralTsProdOutMax=[]  UngainTsProdOutMin=[]  UngainTsProdOutMax=[]  ClampingZeroOutDataTypeStr=Inherit: Inherit via back propagation  ClampingZeroOutMin=[]  ClampingZeroOutMax=[]  FilterDenConstantOutDataTypeStr=Inherit: Inherit via back propagation  FilterDenConstantOutMin=[]  FilterDenConstantOutMax=[]  PCopyOutDataTypeStr=Inherit: Inherit via back propagation  PCopyOutMin=[]  PCopyOutMax=[]  NCopyOutDataTypeStr=Inherit: Inherit via back propagation  NCopyOutMin=[]  NCopyOutMax=[]  IntegratorContinuousStateAttributes=''  IntegratorStateMustResolveToSignalObject=off  IntegratorRTWStateStorageClass=Auto  FilterContinuousStateAttributes=''  FilterStateMustResolveToSignalObject=off  FilterRTWStateStorageClass=Auto  ParallelPVariant=InternalParameters  IdealPVariant=Disabled  IVariant=InternalParameters  DVariant=InternalParameters  IntegratorVariant=Continuous  SatVariant=Enabled  AWVariant=BackCalculation  PCopyVariant=Disabled  TRVariant=Disabled  FdbkBlocksVariant=Forward  IdealPFdbkVariant=Disabled  SatFdbkVariant=Disabled  DerivativeFilterVariant=ContFilter  NVariant=InternalParameters  NCopyVariant=Disabled  FilterICVariant=InternalICsFilter  IntegratorICVariant=InternalICs  ExternalResetVariant=Disabled  TRSumVariant=Passthrough  SumFdbkVariant=Disabled  SumVariant=Sum_PID  TsampFilterVariant=InternalTs  TsampNgainVariant=Passthrough  TsampIntegralVariant=Disabled_SignalSpec  ExternalSaturationOutDataTypeStr=Inherit: Same as second input  DerivativeSourceVariant=ErrorSignal  PreIntVariant=InternalPreInt
  Sum : Sum  Inputs=|+-
  To Workspace : ToWorkspace  VariableName=ALT  SaveFormat=Timeseries  SampleTime=-1
  Theta_ref : Outport
  wires:
  Altitude Ref/1 -> Mux/1, Sum/1
  PID Controller/1 -> Add4/1
  Add4/1 -> Theta_ref/1
  Constant4/1 -> Add4/2
  Sum/1 -> PID Controller/1
  Altitude measured/1 -> Mux/2, Sum/2
  Mux/1 -> To Workspace/1

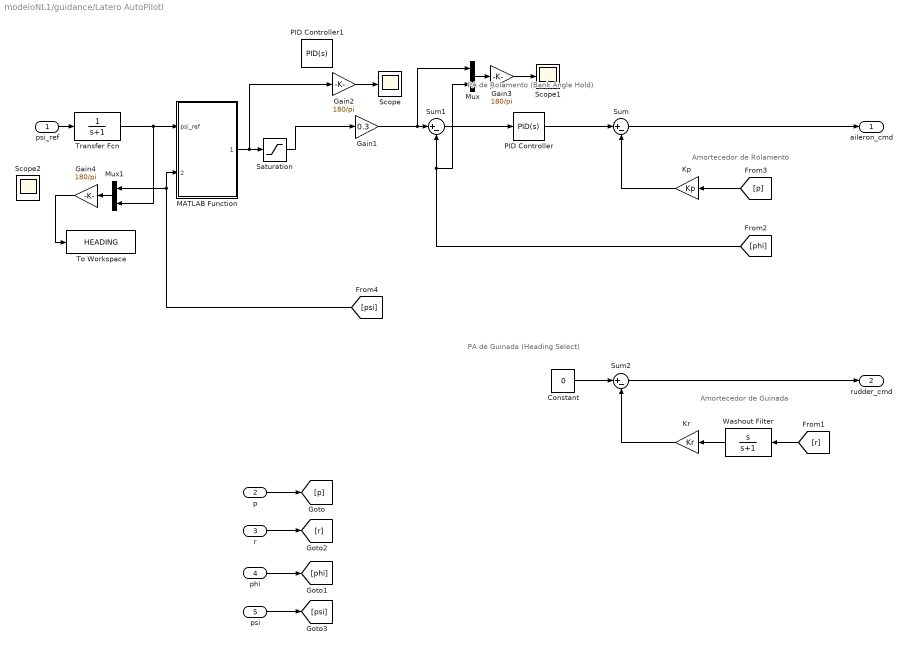
== system modeloNL1/guidance/Latero AutoPilotl ==
  note: PA de Rolamento (Bank Angle Hold)
  note: Amortecedor de Rolamento
  note: Amortecedor de Guinada
  note: PA de Guinada (Heading Select)
  psi_ref : Inport
  p : Inport  Port=2
  r : Inport  Port=3
  phi : Inport  Port=4
  psi : Inport  Port=5
  Constant : Constant  Value=0
  Gain1 : Gain  Gain=0.3
  Gain2 : Gain  Gain=180/pi
  Gain3 : Gain  Gain=180/pi
  Gain4 : Gain  Gain=180/pi
  Kp : Gain  Gain=Kp
  Kr : Gain  Gain=Kr
  MATLAB Function : MATLAB Function  TreatAsAtomicUnit=on
  Mux : Mux  Inputs=2
  Mux1 : Mux  Inputs=2
  PID Controller : slpidlib/PID Controller  Controller=PID  Form=Parallel  TimeDomain=Continuous-time  UseExternalTs=off  SampleTime=-1  IntegratorMethod=Forward Euler  FilterMethod=Forward Euler  ControllerParametersSource=internal  P=C_phi.Kp  I=C_phi.Ki  UseKiTs=off  D=C_phi.Kd  UseExternalDerivativeSource=off  N=C_phi.N  UseFilter=on  TunerSelectOption=Transfer Function Based (PID Tuner App)  InitialConditionSource=internal  InitialConditionForIntegrator=0  InitialConditionForFilter=0  DifferentiatorICPrevScaledInput=0  ExternalReset=none  TrackingMode=off  Kt=1  LimitOutput=on  SatLimitsSource=internal  UpperSaturationLimit=0.43  LowerSaturationLimit=-0.43  LinearizeAsGain=on  AntiWindupMode=back-calculation  Kb=1  LimitIntegrator=off  UpperIntegratorSaturationLimit=inf  LowerIntegratorSaturationLimit=-inf  POutMin=[]  POutMax=[]  IOutMin=[]  IOutMax=[]  DOutMin=[]  DOutMax=[]  NOutMin=[]  NOutMax=[]  SumOutMin=[]  SumOutMax=[]  SaturationOutMin=[]  SaturationOutMax=[]  PParamMin=[]  PParamMax=[]  IParamMin=[]  IParamMax=[]  DParamMin=[]  DParamMax=[]  NParamMin=[]  NParamMax=[]  KbParamMin=[]  KbParamMax=[]  KtParamMin=[]  KtParamMax=[]  KbOutMin=[]  KbOutMax=[]  KtOutMin=[]  KtOutMax=[]  IntegratorOutMin=[]  IntegratorOutMax=[]  FilterOutMin=[]  FilterOutMax=[]  SumI1OutMin=[]  SumI1OutMax=[]  SumI2OutMin=[]  SumI2OutMax=[]  SumI3OutMin=[]  SumI3OutMax=[]  SumI4OutMin=[]  SumI4OutMax=[]  SumDOutMin=[]  SumDOutMax=[]  DifferentiatorOutMin=[]  DifferentiatorOutMax=[]  FilterDiffOutCoefMin=[]  FilterDiffOutCoefMax=[]  ReciprocalOutMin=[]  ReciprocalOutMax=[]  SumDenOutMin=[]  SumDenOutMax=[]  SumNumOutMin=[]  SumNumOutMax=[]  DivideOutMin=[]  DivideOutMax=[]  UdiffTsProdOutMin=[]  UdiffTsProdOutMax=[]  NTsProdOutMin=[]  NTsProdOutMax=[]  UintegralTsProdOutMin=[]  UintegralTsProdOutMax=[]  UngainTsProdOutMin=[]  UngainTsProdOutMax=[]  ClampingZeroOutDataTypeStr=Inherit: Inherit via back propagation  ClampingZeroOutMin=[]  ClampingZeroOutMax=[]  FilterDenConstantOutDataTypeStr=Inherit: Inherit via back propagation  FilterDenConstantOutMin=[]  FilterDenConstantOutMax=[]  PCopyOutDataTypeStr=Inherit: Inherit via back propagation  PCopyOutMin=[]  PCopyOutMax=[]  NCopyOutDataTypeStr=Inherit: Inherit via back propagation  NCopyOutMin=[]  NCopyOutMax=[]  IntegratorContinuousStateAttributes=''  IntegratorStateMustResolveToSignalObject=off  IntegratorRTWStateStorageClass=Auto  FilterContinuousStateAttributes=''  FilterStateMustResolveToSignalObject=off  FilterRTWStateStorageClass=Auto  ParallelPVariant=InternalParameters  IdealPVariant=Disabled  IVariant=InternalParameters  DVariant=InternalParameters  IntegratorVariant=Continuous  SatVariant=Enabled  AWVariant=BackCalculation  PCopyVariant=Disabled  TRVariant=Disabled  FdbkBlocksVariant=Forward  IdealPFdbkVariant=Disabled  SatFdbkVariant=Disabled  DerivativeFilterVariant=ContFilter  NVariant=InternalParameters  NCopyVariant=Disabled  FilterICVariant=InternalICsFilter  IntegratorICVariant=InternalICs  ExternalResetVariant=Disabled  TRSumVariant=Passthrough  SumFdbkVariant=Disabled  SumVariant=Sum_PID  TsampFilterVariant=InternalTs  TsampNgainVariant=Passthrough  TsampIntegralVariant=Disabled_SignalSpec  ExternalSaturationOutDataTypeStr=Inherit: Same as second input  DerivativeSourceVariant=ErrorSignal  PreIntVariant=InternalPreInt
  PID Controller1 : slpidlib/PID Controller  Controller=PID  Form=Parallel  TimeDomain=Continuous-time  UseExternalTs=off  SampleTime=-1  IntegratorMethod=Forward Euler  FilterMethod=Forward Euler  ControllerParametersSource=internal  P=2.5  I=0  UseKiTs=off  D=0  UseExternalDerivativeSource=off  N=100  UseFilter=on  TunerSelectOption=Transfer Function Based (PID Tuner App)  InitialConditionSource=internal  InitialConditionForIntegrator=0  InitialConditionForFilter=0  DifferentiatorICPrevScaledInput=0  ExternalReset=none  TrackingMode=off  Kt=1  LimitOutput=off  SatLimitsSource=internal  UpperSaturationLimit=inf  LowerSaturationLimit=-inf  LinearizeAsGain=on  AntiWindupMode=none  Kb=1  LimitIntegrator=off  UpperIntegratorSaturationLimit=inf  LowerIntegratorSaturationLimit=-inf  POutMin=[]  POutMax=[]  IOutMin=[]  IOutMax=[]  DOutMin=[]  DOutMax=[]  NOutMin=[]  NOutMax=[]  SumOutMin=[]  SumOutMax=[]  SaturationOutMin=[]  SaturationOutMax=[]  PParamMin=[]  PParamMax=[]  IParamMin=[]  IParamMax=[]  DParamMin=[]  DParamMax=[]  NParamMin=[]  NParamMax=[]  KbParamMin=[]  KbParamMax=[]  KtParamMin=[]  KtParamMax=[]  KbOutMin=[]  KbOutMax=[]  KtOutMin=[]  KtOutMax=[]  IntegratorOutMin=[]  IntegratorOutMax=[]  FilterOutMin=[]  FilterOutMax=[]  SumI1OutMin=[]  SumI1OutMax=[]  SumI2OutMin=[]  SumI2OutMax=[]  SumI3OutMin=[]  SumI3OutMax=[]  SumI4OutMin=[]  SumI4OutMax=[]  SumDOutMin=[]  SumDOutMax=[]  DifferentiatorOutMin=[]  DifferentiatorOutMax=[]  FilterDiffOutCoefMin=[]  FilterDiffOutCoefMax=[]  ReciprocalOutMin=[]  ReciprocalOutMax=[]  SumDenOutMin=[]  SumDenOutMax=[]  SumNumOutMin=[]  SumNumOutMax=[]  DivideOutMin=[]  DivideOutMax=[]  UdiffTsProdOutMin=[]  UdiffTsProdOutMax=[]  NTsProdOutMin=[]  NTsProdOutMax=[]  UintegralTsProdOutMin=[]  UintegralTsProdOutMax=[]  UngainTsProdOutMin=[]  UngainTsProdOutMax=[]  ClampingZeroOutDataTypeStr=Inherit: Inherit via back propagation  ClampingZeroOutMin=[]  ClampingZeroOutMax=[]  FilterDenConstantOutDataTypeStr=Inherit: Inherit via back propagation  FilterDenConstantOutMin=[]  FilterDenConstantOutMax=[]  PCopyOutDataTypeStr=Inherit: Inherit via back propagation  PCopyOutMin=[]  PCopyOutMax=[]  NCopyOutDataTypeStr=Inherit: Inherit via back propagation  NCopyOutMin=[]  NCopyOutMax=[]  IntegratorContinuousStateAttributes=''  IntegratorStateMustResolveToSignalObject=off  IntegratorRTWStateStorageClass=Auto  FilterContinuousStateAttributes=''  FilterStateMustResolveToSignalObject=off  FilterRTWStateStorageClass=Auto  ParallelPVariant=InternalParameters  IdealPVariant=Disabled  IVariant=InternalParameters  DVariant=InternalParameters  IntegratorVariant=Continuous  SatVariant=Disabled  AWVariant=Passthrough  PCopyVariant=Disabled  TRVariant=Disabled  FdbkBlocksVariant=Forward  IdealPFdbkVariant=Disabled  SatFdbkVariant=Disabled  DerivativeFilterVariant=ContFilter  NVariant=InternalParameters  NCopyVariant=Disabled  FilterICVariant=InternalICsFilter  IntegratorICVariant=InternalICs  ExternalResetVariant=Disabled  TRSumVariant=Passthrough  SumFdbkVariant=Disabled  SumVariant=Sum_PID  TsampFilterVariant=InternalTs  TsampNgainVariant=Passthrough  TsampIntegralVariant=Disabled_SignalSpec  ExternalSaturationOutDataTypeStr=Inherit: Same as second input  DerivativeSourceVariant=ErrorSignal  PreIntVariant=InternalPreInt
  Saturation : Saturate  UpperLimit=1.0  LowerLimit=-1.0
  Scope : Scope
      settings: ActiveDisplayYMinimum=-3.05499  ActiveDisplayYMaximum=27.49487  DataLoggingVariableName=ScopeData3
  Scope1 : Scope
      settings: ActiveDisplayYMinimum=-0.54177  ActiveDisplayYMaximum=4.86179  DataLoggingVariableName=ScopeData4
  Scope2 : Scope
      settings: ActiveDisplayYMinimum=-1  ActiveDisplayYMaximum=1  DataLoggingVariableName=ScopeData5
  Sum : Sum  Inputs=|+-
  Sum1 : Sum  Inputs=|+-
  Sum2 : Sum  Inputs=|+-
  To Workspace : ToWorkspace  VariableName=HEADING  SampleTime=-1
  Transfer Fcn : TransferFcn  Denominator=[1 1]
  Washout Filter : TransferFcn  Numerator=[1 0]  Denominator=[1 1]
  aileron_cmd : Outport
  rudder_cmd : Outport  Port=2
  wires:
  Sum/1 -> aileron_cmd/1
  [p] -> Kp/1
  [phi] -> Mux/2, Sum1/2
  Kp/1 -> Sum/2
  PID Controller/1 -> Sum/1
  p/1 -> [p]
  [r] -> Washout Filter/1
  Kr/1 -> Sum2/2
  r/1 -> [r]
  Washout Filter/1 -> Kr/1
  phi/1 -> [phi]
  psi/1 -> [psi]
  Sum2/1 -> rudder_cmd/1
  Constant/1 -> Sum2/1
  Gain1/1 -> Mux/1, Sum1/1
  psi_ref/1 -> Transfer Fcn/1
  [psi] -> Mux1/1, MATLAB Function/2(psi_atual)
  MATLAB Function/1(erro_psi) -> Gain2/1, Saturation/1
  Gain2/1 -> Scope/1
  Saturation/1 -> Gain1/1
  Gain3/1 -> Scope1/1
  Sum1/1 -> PID Controller/1
  Mux/1 -> Gain3/1
  Mux1/1 -> Gain4/1
  Transfer Fcn/1 -> Mux1/2, MATLAB Function/1(psi_ref)
  Gain4/1 -> To Workspace/1

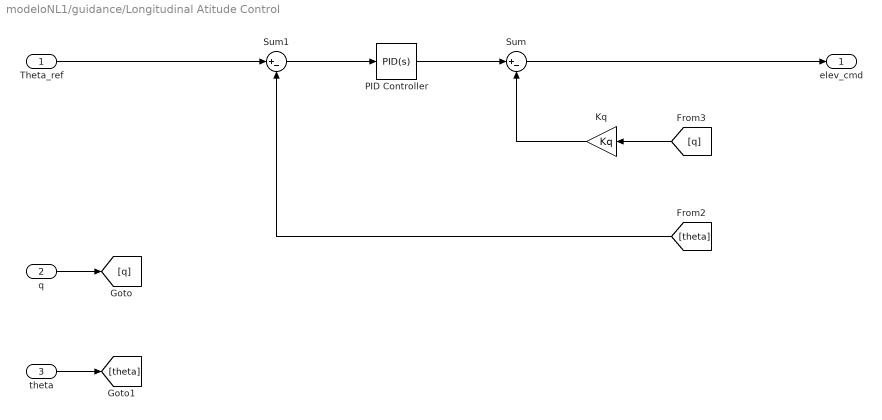
== system modeloNL1/guidance/Longitudinal Atitude Control ==
  Theta_ref : Inport
  q : Inport  Port=2
  theta : Inport  Port=3
  Kq : Gain  Gain=Kq
  PID Controller : slpidlib/PID Controller  Controller=PID  Form=Parallel  TimeDomain=Continuous-time  UseExternalTs=off  SampleTime=-1  IntegratorMethod=Forward Euler  FilterMethod=Forward Euler  ControllerParametersSource=internal  P=C_theta.Kp  I=C_theta.Ki  UseKiTs=off  D=C_theta.Kd  UseExternalDerivativeSource=off  N=C_theta.N  UseFilter=on  TunerSelectOption=Transfer Function Based (PID Tuner App)  InitialConditionSource=internal  InitialConditionForIntegrator=0  InitialConditionForFilter=0  DifferentiatorICPrevScaledInput=0  ExternalReset=none  TrackingMode=off  Kt=1  LimitOutput=on  SatLimitsSource=internal  UpperSaturationLimit=inf  LowerSaturationLimit=-inf  LinearizeAsGain=on  AntiWindupMode=back-calculation  Kb=1  LimitIntegrator=off  UpperIntegratorSaturationLimit=inf  LowerIntegratorSaturationLimit=-inf  POutMin=[]  POutMax=[]  IOutMin=[]  IOutMax=[]  DOutMin=[]  DOutMax=[]  NOutMin=[]  NOutMax=[]  SumOutMin=[]  SumOutMax=[]  SaturationOutMin=[]  SaturationOutMax=[]  PParamMin=[]  PParamMax=[]  IParamMin=[]  IParamMax=[]  DParamMin=[]  DParamMax=[]  NParamMin=[]  NParamMax=[]  KbParamMin=[]  KbParamMax=[]  KtParamMin=[]  KtParamMax=[]  KbOutMin=[]  KbOutMax=[]  KtOutMin=[]  KtOutMax=[]  IntegratorOutMin=[]  IntegratorOutMax=[]  FilterOutMin=[]  FilterOutMax=[]  SumI1OutMin=[]  SumI1OutMax=[]  SumI2OutMin=[]  SumI2OutMax=[]  SumI3OutMin=[]  SumI3OutMax=[]  SumI4OutMin=[]  SumI4OutMax=[]  SumDOutMin=[]  SumDOutMax=[]  DifferentiatorOutMin=[]  DifferentiatorOutMax=[]  FilterDiffOutCoefMin=[]  FilterDiffOutCoefMax=[]  ReciprocalOutMin=[]  ReciprocalOutMax=[]  SumDenOutMin=[]  SumDenOutMax=[]  SumNumOutMin=[]  SumNumOutMax=[]  DivideOutMin=[]  DivideOutMax=[]  UdiffTsProdOutMin=[]  UdiffTsProdOutMax=[]  NTsProdOutMin=[]  NTsProdOutMax=[]  UintegralTsProdOutMin=[]  UintegralTsProdOutMax=[]  UngainTsProdOutMin=[]  UngainTsProdOutMax=[]  ClampingZeroOutDataTypeStr=Inherit: Inherit via back propagation  ClampingZeroOutMin=[]  ClampingZeroOutMax=[]  FilterDenConstantOutDataTypeStr=Inherit: Inherit via back propagation  FilterDenConstantOutMin=[]  FilterDenConstantOutMax=[]  PCopyOutDataTypeStr=Inherit: Inherit via back propagation  PCopyOutMin=[]  PCopyOutMax=[]  NCopyOutDataTypeStr=Inherit: Inherit via back propagation  NCopyOutMin=[]  NCopyOutMax=[]  IntegratorContinuousStateAttributes=''  IntegratorStateMustResolveToSignalObject=off  IntegratorRTWStateStorageClass=Auto  FilterContinuousStateAttributes=''  FilterStateMustResolveToSignalObject=off  FilterRTWStateStorageClass=Auto  ParallelPVariant=InternalParameters  IdealPVariant=Disabled  IVariant=InternalParameters  DVariant=InternalParameters  IntegratorVariant=Continuous  SatVariant=Enabled  AWVariant=BackCalculation  PCopyVariant=Disabled  TRVariant=Disabled  FdbkBlocksVariant=Forward  IdealPFdbkVariant=Disabled  SatFdbkVariant=Disabled  DerivativeFilterVariant=ContFilter  NVariant=InternalParameters  NCopyVariant=Disabled  FilterICVariant=InternalICsFilter  IntegratorICVariant=InternalICs  ExternalResetVariant=Disabled  TRSumVariant=Passthrough  SumFdbkVariant=Disabled  SumVariant=Sum_PID  TsampFilterVariant=InternalTs  TsampNgainVariant=Passthrough  TsampIntegralVariant=Disabled_SignalSpec  ExternalSaturationOutDataTypeStr=Inherit: Same as second input  DerivativeSourceVariant=ErrorSignal  PreIntVariant=InternalPreInt
  Sum : Sum  Inputs=|+-
  Sum1 : Sum  Inputs=|+-
  elev_cmd : Outport
  wires:
  Sum1/1 -> PID Controller/1
  Sum/1 -> elev_cmd/1
  Theta_ref/1 -> Sum1/1
  [q] -> Kq/1
  [theta] -> Sum1/2
  Kq/1 -> Sum/2
  PID Controller/1 -> Sum/1
  theta/1 -> [theta]
  q/1 -> [q]

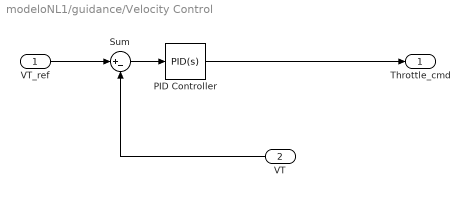
== system modeloNL1/guidance/Velocity Control ==
  VT_ref : Inport
  VT : Inport  Port=2
  PID Controller : slpidlib/PID Controller  Controller=PID  Form=Parallel  TimeDomain=Continuous-time  UseExternalTs=off  SampleTime=-1  IntegratorMethod=Forward Euler  FilterMethod=Forward Euler  ControllerParametersSource=internal  P=C_vel.Kp  I=C_vel.Ki  UseKiTs=off  D=C_vel.Kd  UseExternalDerivativeSource=off  N=C_vel.N  UseFilter=on  TunerSelectOption=Transfer Function Based (PID Tuner App)  InitialConditionSource=internal  InitialConditionForIntegrator=0  InitialConditionForFilter=0  DifferentiatorICPrevScaledInput=0  ExternalReset=none  TrackingMode=off  Kt=1  LimitOutput=on  SatLimitsSource=internal  UpperSaturationLimit=inf  LowerSaturationLimit=-inf  LinearizeAsGain=on  AntiWindupMode=back-calculation  Kb=1  LimitIntegrator=off  UpperIntegratorSaturationLimit=inf  LowerIntegratorSaturationLimit=-inf  POutMin=[]  POutMax=[]  IOutMin=[]  IOutMax=[]  DOutMin=[]  DOutMax=[]  NOutMin=[]  NOutMax=[]  SumOutMin=[]  SumOutMax=[]  SaturationOutMin=[]  SaturationOutMax=[]  PParamMin=[]  PParamMax=[]  IParamMin=[]  IParamMax=[]  DParamMin=[]  DParamMax=[]  NParamMin=[]  NParamMax=[]  KbParamMin=[]  KbParamMax=[]  KtParamMin=[]  KtParamMax=[]  KbOutMin=[]  KbOutMax=[]  KtOutMin=[]  KtOutMax=[]  IntegratorOutMin=[]  IntegratorOutMax=[]  FilterOutMin=[]  FilterOutMax=[]  SumI1OutMin=[]  SumI1OutMax=[]  SumI2OutMin=[]  SumI2OutMax=[]  SumI3OutMin=[]  SumI3OutMax=[]  SumI4OutMin=[]  SumI4OutMax=[]  SumDOutMin=[]  SumDOutMax=[]  DifferentiatorOutMin=[]  DifferentiatorOutMax=[]  FilterDiffOutCoefMin=[]  FilterDiffOutCoefMax=[]  ReciprocalOutMin=[]  ReciprocalOutMax=[]  SumDenOutMin=[]  SumDenOutMax=[]  SumNumOutMin=[]  SumNumOutMax=[]  DivideOutMin=[]  DivideOutMax=[]  UdiffTsProdOutMin=[]  UdiffTsProdOutMax=[]  NTsProdOutMin=[]  NTsProdOutMax=[]  UintegralTsProdOutMin=[]  UintegralTsProdOutMax=[]  UngainTsProdOutMin=[]  UngainTsProdOutMax=[]  ClampingZeroOutDataTypeStr=Inherit: Inherit via back propagation  ClampingZeroOutMin=[]  ClampingZeroOutMax=[]  FilterDenConstantOutDataTypeStr=Inherit: Inherit via back propagation  FilterDenConstantOutMin=[]  FilterDenConstantOutMax=[]  PCopyOutDataTypeStr=Inherit: Inherit via back propagation  PCopyOutMin=[]  PCopyOutMax=[]  NCopyOutDataTypeStr=Inherit: Inherit via back propagation  NCopyOutMin=[]  NCopyOutMax=[]  IntegratorContinuousStateAttributes=''  IntegratorStateMustResolveToSignalObject=off  IntegratorRTWStateStorageClass=Auto  FilterContinuousStateAttributes=''  FilterStateMustResolveToSignalObject=off  FilterRTWStateStorageClass=Auto  ParallelPVariant=InternalParameters  IdealPVariant=Disabled  IVariant=InternalParameters  DVariant=InternalParameters  IntegratorVariant=Continuous  SatVariant=Enabled  AWVariant=BackCalculation  PCopyVariant=Disabled  TRVariant=Disabled  FdbkBlocksVariant=Forward  IdealPFdbkVariant=Disabled  SatFdbkVariant=Disabled  DerivativeFilterVariant=ContFilter  NVariant=InternalParameters  NCopyVariant=Disabled  FilterICVariant=InternalICsFilter  IntegratorICVariant=InternalICs  ExternalResetVariant=Disabled  TRSumVariant=Passthrough  SumFdbkVariant=Disabled  SumVariant=Sum_PID  TsampFilterVariant=InternalTs  TsampNgainVariant=Passthrough  TsampIntegralVariant=Disabled_SignalSpec  ExternalSaturationOutDataTypeStr=Inherit: Same as second input  DerivativeSourceVariant=ErrorSignal  PreIntVariant=InternalPreInt
  Sum : Sum  Inputs=|+-
  Throttle_cmd : Outport
  wires:
  VT/1 -> Sum/2
  PID Controller/1 -> Throttle_cmd/1
  VT_ref/1 -> Sum/1
  Sum/1 -> PID Controller/1

== matlab function modeloNL1/guidance/Latero AutoPilotl/MATLAB Function ==
  data: psi_ref input; erro_psi output; psi_atual input
function erro_psi = calc_erro_proa(psi_ref, psi_atual)
    % Calcula a diferença simples
    diff = psi_ref - psi_atual;
    
    % Normaliza para o intervalo [-pi, +pi]
    % Isso garante que o avião sempre vire pelo lado mais curto.
    % Exemplo: Se quero ir para 350 mas estou em 10, o erro é -20, não +340.
    
    erro_psi = mod(diff + pi, 2*pi) - pi;
end
